simulink model "mod_pv"  (R2019b)
settings: Solver=ode1  StartTime=0.0  StopTime=1  FixedStep=1e-4  RelTol=1e-3
libraries: simulink x1
settings Model: Creator=flocment  LastModifiedBy=flocment

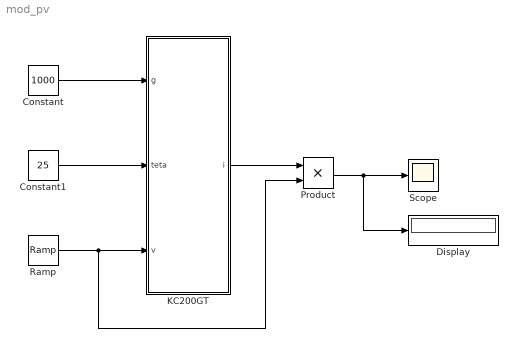
== system mod_pv ==
  Constant : Constant  Value=1000
  Constant1 : Constant  Value=25
  Display : Display
  KC200GT : Subsystem
  Product : Product
  Ramp : simulink/Sources/Ramp  slope=(40-0)/(1-0)  start=0  InitialOutput=0
  Scope : Scope
  wires:
  Constant/1 -> KC200GT/1(g)
  Constant1/1 -> KC200GT/2(teta)
  Ramp/1 -> Product/2, KC200GT/3(v)
  KC200GT/1(i) -> Product/1
  Product/1 -> Display/1, Scope/1

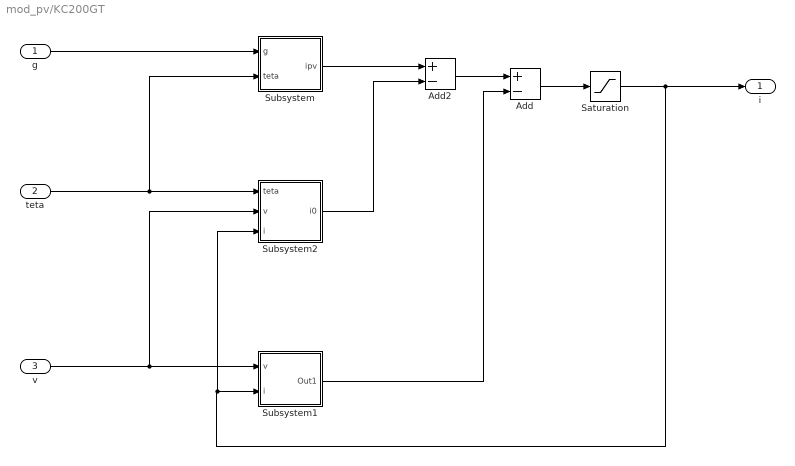
== system mod_pv/KC200GT ==
  g : Inport
  teta : Inport  Port=2
  v : Inport  Port=3
  Add : Sum  Inputs=+-
  Add2 : Sum  Inputs=+-
  Saturation : Saturate  UpperLimit=inf  LowerLimit=0
  Subsystem : Subsystem
  Subsystem1 : Subsystem
  Subsystem2 : Subsystem
  i : Outport
  wires:
  Subsystem/1(ipv) -> Add2/1
  g/1 -> Subsystem/1(g)
  Add2/1 -> Add/1
  Add/1 -> Saturation/1
  teta/1 -> Subsystem/2(teta), Subsystem2/1(teta)
  v/1 -> Subsystem2/2(v), Subsystem1/1(v)
  Saturation/1 -> i/1, Subsystem2/3(i), Subsystem1/2(i)
  Subsystem1/1(Out1) -> Add/2
  Subsystem2/1(i0) -> Add2/2

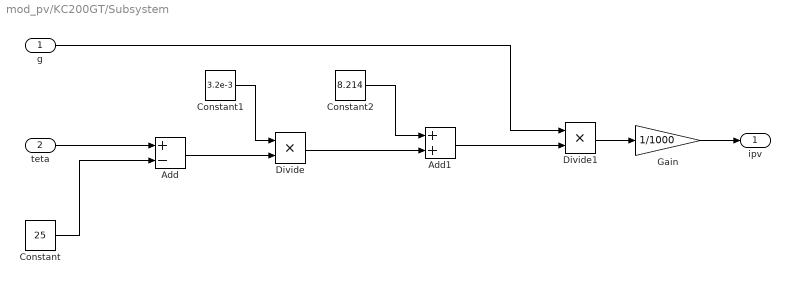
== system mod_pv/KC200GT/Subsystem ==
  g : Inport
  teta : Inport  Port=2
  Add : Sum  Inputs=+-
  Add1 : Sum
  Constant : Constant  Value=25
  Constant1 : Constant  Value=3.2e-3
  Constant2 : Constant  Value=8.214
  Divide : Product  Inputs=**
  Divide1 : Product  Inputs=**
  Gain : Gain  Gain=1/1000
  ipv : Outport
  wires:
  Constant1/1 -> Divide/1
  Constant2/1 -> Add1/1
  Constant/1 -> Add/2
  Divide1/1 -> Gain/1
  Add1/1 -> Divide1/2
  g/1 -> Divide1/1
  Divide/1 -> Add1/2
  teta/1 -> Add/1
  Add/1 -> Divide/2
  Gain/1 -> ipv/1

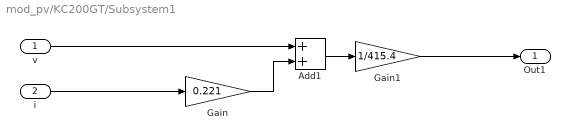
== system mod_pv/KC200GT/Subsystem1 ==
  v : Inport
  i : Inport  Port=2
  Add1 : Sum
  Gain : Gain  Gain=0.221
  Gain1 : Gain  Gain=1/415.4
  Out1 : Outport
  wires:
  Gain1/1 -> Out1/1
  Gain/1 -> Add1/2
  Add1/1 -> Gain1/1
  i/1 -> Gain/1
  v/1 -> Add1/1

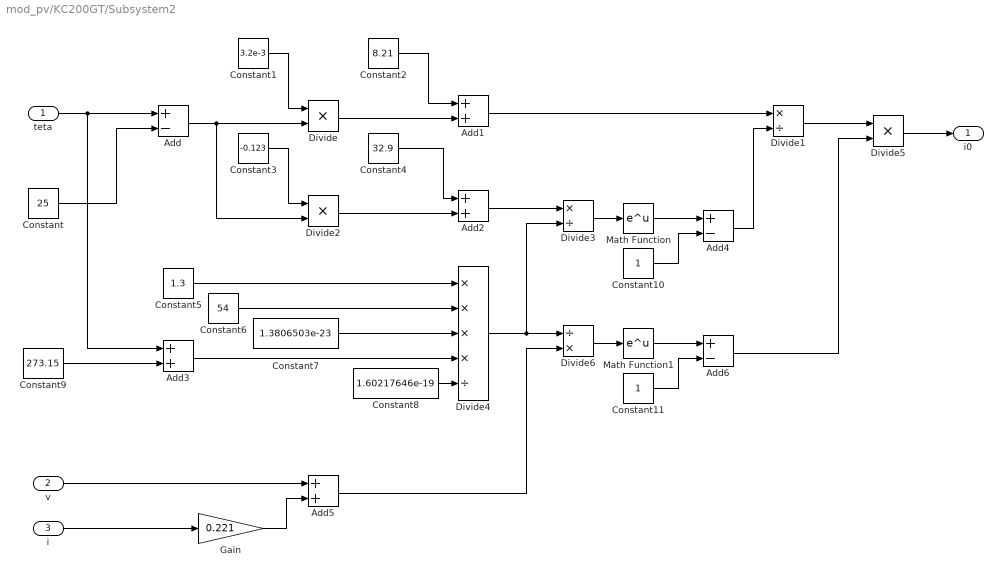
== system mod_pv/KC200GT/Subsystem2 ==
  teta : Inport
  v : Inport  Port=2
  i : Inport  Port=3
  Add : Sum  Inputs=+-
  Add{1..3,5} (4 alike) : Sum
  Add4 : Sum  Inputs=+-
  Add6 : Sum  Inputs=+-
  Constant : Constant  Value=25
  Constant1 : Constant  Value=3.2e-3
  Constant10 : Constant
  Constant11 : Constant
  Constant2 : Constant  Value=8.21
  Constant3 : Constant  Value=-0.123
  Constant4 : Constant  Value=32.9
  Constant5 : Constant  Value=1.3
  Constant6 : Constant  Value=54
  Constant7 : Constant  Value=1.3806503e-23
  Constant8 : Constant  Value=1.60217646e-19
  Constant9 : Constant  Value=273.15
  Divide : Product  Inputs=**
  Divide1 : Product  Inputs=*/
  Divide2 : Product  Inputs=**
  Divide3 : Product  Inputs=*/
  Divide4 : Product  Inputs=****/
  Divide5 : Product  Inputs=**
  Divide6 : Product  Inputs=/*
  Gain : Gain  Gain=0.221
  Math Function : Math  SignedPower=off  SaturateOnIntegerOverflow=on
  Math Function1 : Math  SignedPower=off  SaturateOnIntegerOverflow=on
  i0 : Outport
  wires:
  Constant1/1 -> Divide/1
  Constant2/1 -> Add1/1
  Constant/1 -> Add/2
  Divide/1 -> Add1/2
  Add/1 -> Divide2/2, Divide/2
  Add1/1 -> Divide1/1
  Constant3/1 -> Divide2/1
  Constant4/1 -> Add2/1
  Divide2/1 -> Add2/2
  Add2/1 -> Divide3/1
  Constant5/1 -> Divide4/1
  Divide4/1 -> Divide6/1, Divide3/2
  Constant6/1 -> Divide4/2
  Constant7/1 -> Divide4/3
  Constant8/1 -> Divide4/5
  Add3/1 -> Divide4/4
  teta/1 -> Add3/1, Add/1
  Constant9/1 -> Add3/2
  Divide3/1 -> Math Function/1
  Math Function/1 -> Add4/1
  Constant10/1 -> Add4/2
  Divide1/1 -> Divide5/1
  Gain/1 -> Add5/2
  Add5/1 -> Divide6/2
  i/1 -> Gain/1
  v/1 -> Add5/1
  Math Function1/1 -> Add6/1
  Constant11/1 -> Add6/2
  Divide6/1 -> Math Function1/1
  Add6/1 -> Divide5/2
  Divide5/1 -> i0/1
  Add4/1 -> Divide1/2
